simulink model "MPC_sim"  (R2024b)
settings: Solver=FixedStepAuto  StartTime=0.0  StopTime=inf  FixedStep=0.001  RelTol=1e-3  EnableMultiTasking=on
values from neighbouring files (symbols this model uses):
  Ts = 0.01    [MPC.m]    (also in mpc3D.m)
libraries: mpclib x2, px4Sensorslib x2, px4Peripheralslib x1
settings Model: SimulationMode=external  ExtModeTrigDuration=10  Creator=ArriGE66  LastModifiedBy=xippa
settings SolverCC: PositivePriorityOrder=on
settings OptimizationCC: EnhancedBackFolding=on  PassReuseOutputArgsAs=Individual arguments  ZeroExternalMemoryAtStartup=off  ZeroInternalMemoryAtStartup=off  MaxStackSize=64  OptimizeBlockOrder=speed  DifferentSizesBufferReuse=on  OptimizationCustomize=off  EfficientTunableParamExpr=on
settings DebuggingCC: ParameterTunabilityLossMsg=error
settings HardwareCC: ProdBitPerPointer=32  ProdBitPerSizeT=32  ProdBitPerPtrDiffT=32  ProdLargestAtomicInteger=Long  ProdLargestAtomicFloat=Double  ProdWordSize=32  ProdLongLongMode=on  ProdHWDeviceType=ARM Compatible->ARM Cortex
settings SFSimCC: MATLABDynamicMemAlloc=off  SimTargetLang=C++
settings RTWCC: Description=Embedded Coder  SystemTargetFile=ert.tlc  HardwareBoard=PX4 Cube Orange  TemplateMakefile=ert_default_tmf  Toolchain=GNU Tools for PX4 Autopilots  TargetLang=C++  GPUComputeCapability=3.5
settings CodeAppCC: ForceParamTrailComments=on  IgnoreCustomStorageClasses=off  OperatorAnnotations=on  SimulinkDataObjDesc=on  SFDataObjDesc=on  InsertBlockDesc=on
settings ERTTargetCC: SupportVariableSizeSignals=on  ExtMode=on  ExtModeTransport=3  ExtModeStaticAlloc=on  ExtModeStaticAllocSize=1024  ExtModeMexFile=ext_xcp  ExtModeMexArgs=1 COM10 3000000  ExtModeIntrfLevel=Level2 - Open  InlinedParameterPlacement=Hierarchical  DynamicArrayContainerType=coder::array

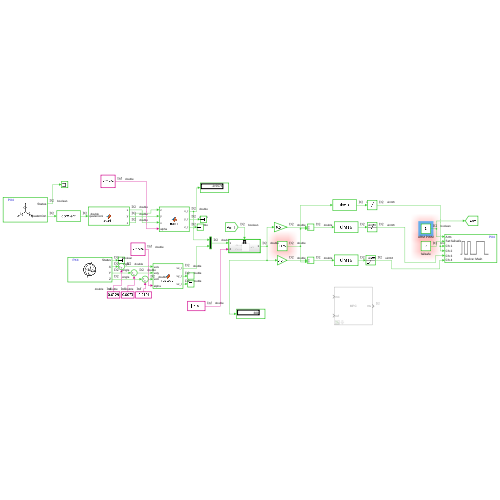
[thumbnail: Simulink's stored preview of the top-level diagram]
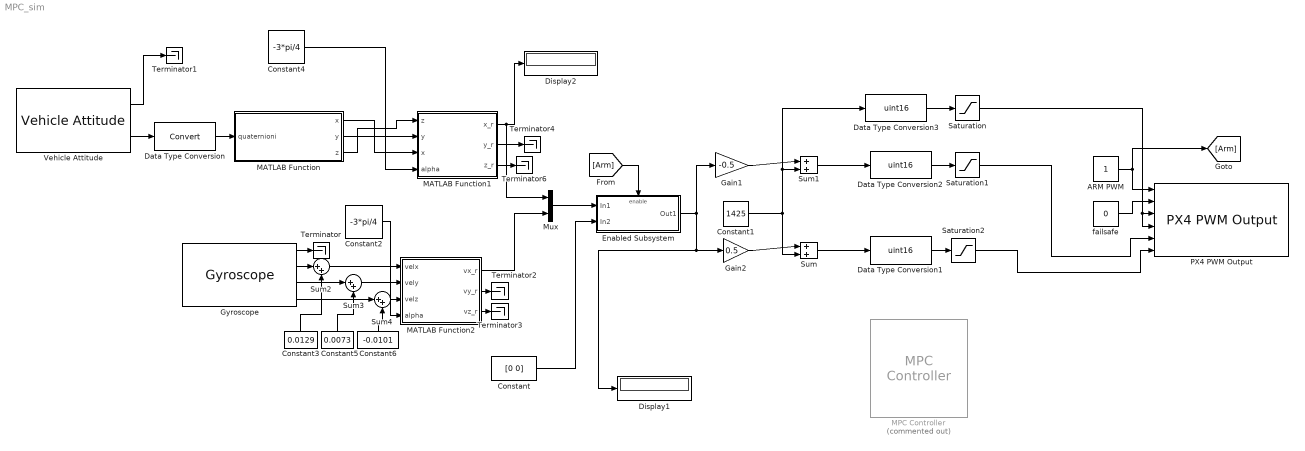
== system MPC_sim ==
  ARM PWM : Constant  OutDataTypeStr=boolean  SampleTime=Ts
  Constant : Constant  Value=[0 0]
  Constant1 : Constant  Value=1425  SampleTime=Ts
  Constant2 : Constant  Value=-3*pi/4
  Constant3 : Constant  Value=0.0129
  Constant4 : Constant  Value=-3*pi/4
  Constant5 : Constant  Value=0.0073
  Constant6 : Constant  Value=-0.0101
  Data Type Conversion : DataTypeConversion  SaturateOnIntegerOverflow=off  RndMeth=Floor
  Data Type Conversion1 : DataTypeConversion  OutDataTypeStr=uint16  SaturateOnIntegerOverflow=off  RndMeth=Floor
  Data Type Conversion2 : DataTypeConversion  OutDataTypeStr=uint16  SaturateOnIntegerOverflow=off  RndMeth=Floor
  Data Type Conversion3 : DataTypeConversion  OutDataTypeStr=uint16  SaturateOnIntegerOverflow=off  RndMeth=Floor
  Display1 : Display
  Display2 : Display
  Enabled Subsystem : Subsystem  TreatAsAtomicUnit=on
  Gain1 : Gain  Gain=-0.5
  Gain2 : Gain  Gain=0.5
  Gyroscope : px4Sensorslib/Gyroscope  uorbTimeStamp=off  BlockingMode=off  BlockTimeout=1e-3  sampleTime=Ts
  MATLAB Function : MATLAB Function  TreatAsAtomicUnit=on
  MATLAB Function1 : MATLAB Function  TreatAsAtomicUnit=on
  MATLAB Function2 : MATLAB Function  TreatAsAtomicUnit=on
  MPC Controller : mpclib/MPC Controller  Commented=on  SCDEnableBlockLinearizationSpecification=on  mpcobj=mpcobj  x0=Init_cond  is_multiple=0  enable_value=0  return_u0=off  updateMPCinCallerWorkspace=on  md_inport=off  mv_inport=off  uref_inport=off  return_cost=off  return_mvseq=off  return_qpstatus=off  return_xseq=off  return_state=off  return_ovseq=off  state_inport=off  umin_inport=off  umax_inport=off  ymin_inport=off  ymax_inport=off  cc_inport=off  ywt_inport=off  uwt_inport=off  duwt_inport=off  rhoeps_inport=off  pm_inport=off  MaximumP=10  HorizonChoice=FixedHorizon  n_ts=0.01  n_p=80  n_mv=1  n_md=0  n_ud=0  n_mo=2  n_uo=0  BlockDataType=double  SampleTimeInherited=off  switch_inport=off
  Mux : Mux  Inputs=2
  PX4 PWM Output : px4Peripheralslib/PX4 PWM Output  pwmDevice=Main  pwmChannel1_=on  pwmChannel2_=on  pwmChannel3_=on  pwmChannel4_=on  pwmChannel5_=off  pwmChannel6_=off  pwmChannel7_=off  pwmChannel8_=off
  Saturation : Saturate  UpperLimit=1800  LowerLimit=1100
  Saturation1 : Saturate  UpperLimit=1800  LowerLimit=1100
  Saturation2 : Saturate  UpperLimit=1800  LowerLimit=1100
  Sum{,1..4} (5 alike) : Sum  Inputs=|++
  Terminator{,1..4,6} (6 alike) : Terminator
  Vehicle Attitude : px4Sensorslib/Vehicle Attitude  rollRate=off  pitchRate=off  yawRate=off  quaternion=on  uorbTimeStamp=off  BlockingMode=off  BlockTimeout=0.001  sampleTime=Ts
  failsafe : Constant  Value=0  OutDataTypeStr=boolean  SampleTime=Ts
  wires:
  Gain1/1 -> Sum1/1
  Gain2/1 -> Sum/1
  Vehicle Attitude/1 -> Terminator1/1
  Vehicle Attitude/2 -> Data Type Conversion/1
  Gyroscope/1 -> Terminator/1
  Gyroscope/3 -> Sum3/1
  Constant2/1 -> MATLAB Function2/4(alpha)
  Gyroscope/2 -> Sum2/1
  Gyroscope/4 -> Sum4/1
  MATLAB Function/1(x) -> MATLAB Function1/3(x)
  MATLAB Function/2(y) -> MATLAB Function1/2(y)
  MATLAB Function/3(z) -> MATLAB Function1/1(z)
  Constant4/1 -> MATLAB Function1/4(alpha)
  Constant1/1 -> Sum1/2, Data Type Conversion3/1, Sum/2
  Sum/1 -> Data Type Conversion1/1
  Sum1/1 -> Data Type Conversion2/1
  Data Type Conversion1/1 -> Saturation2/1
  Data Type Conversion2/1 -> Saturation1/1
  ARM PWM/1 -> PX4 PWM Output/1, [Arm]
  Data Type Conversion3/1 -> Saturation/1
  failsafe/1 -> PX4 PWM Output/2
  MATLAB Function1/1(x_r) -> Display2/1, Mux/1
  MATLAB Function2/1(vx_r) -> Mux/2
  Saturation/1 -> PX4 PWM Output/4, PX4 PWM Output/3
  Saturation2/1 -> PX4 PWM Output/6
  Saturation1/1 -> PX4 PWM Output/5
  Constant5/1 -> Sum3/2
  Constant3/1 -> Sum2/2
  Constant6/1 -> Sum4/2
  Sum2/1 -> MATLAB Function2/1(velx)
  Sum3/1 -> MATLAB Function2/2(vely)
  Sum4/1 -> MATLAB Function2/3(velz)
  MATLAB Function2/2(vy_r) -> Terminator2/1
  MATLAB Function2/3(vz_r) -> Terminator3/1
  MATLAB Function1/2(y_r) -> Terminator4/1
  MATLAB Function1/3(z_r) -> Terminator6/1
  Data Type Conversion/1 -> MATLAB Function/1(quaternioni)
  Mux/1 -> Enabled Subsystem/1(In1)
  Constant/1 -> Enabled Subsystem/2(In2)
  Enabled Subsystem/1(Out1) -> Gain2/1, Display1/1, Gain1/1
  [Arm] -> Enabled Subsystem/Enable

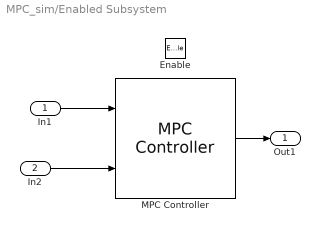
== system MPC_sim/Enabled Subsystem ==
  In1 : Inport
  In2 : Inport  Port=2
  Enable : EnablePort
  MPC Controller : mpclib/MPC Controller  SCDEnableBlockLinearizationSpecification=on  mpcobj=mpcobj  x0=Init_cond  is_multiple=0  enable_value=0  return_u0=off  updateMPCinCallerWorkspace=on  md_inport=off  mv_inport=off  uref_inport=off  return_cost=off  return_mvseq=off  return_qpstatus=off  return_xseq=off  return_state=off  return_ovseq=off  state_inport=off  umin_inport=off  umax_inport=off  ymin_inport=off  ymax_inport=off  cc_inport=off  ywt_inport=off  uwt_inport=off  duwt_inport=off  rhoeps_inport=off  pm_inport=off  MaximumP=10  HorizonChoice=FixedHorizon  n_ts=0.01  n_p=10  n_mv=1  n_md=0  n_ud=0  n_mo=2  n_uo=0  BlockDataType=double  SampleTimeInherited=off  switch_inport=off
  Out1 : Outport
  wires:
  In1/1 -> MPC Controller/1
  In2/1 -> MPC Controller/2
  MPC Controller/1 -> Out1/1

== matlab function MPC_sim/MATLAB Function1 ==
  data: z input; y input; x input; x_r output; alpha input; y_r output; z_r output
function [x_r,y_r,z_r] = ruoto(z,y,x,alpha)
Global_POV = [x y z];
R_z = [cos(alpha), -sin(alpha), 0;
       sin(alpha), cos(alpha), 0;
       0, 0, 1];
LOCALPOV = Global_POV * R_z;
x_r = LOCALPOV(1);
y_r = LOCALPOV(2);
z_r = LOCALPOV(3);
end

== matlab function MPC_sim/MATLAB Function ==
  data: x output; y output; quaternioni input; z output
function [x, y, z] = assetto(quaternioni)
    % Estrazione dei componenti del quaternione
    qw = quaternioni(1);
    qx = quaternioni(2);
    qy = quaternioni(3);
    qz = quaternioni(4);

    % Calcolo degli angoli di Eulero manualmente
    x = atan2(2*(qw*qx + qy*qz), 1 - 2*(qx^2 + qy^2)); % roll
    y = asin(2*(qw*qy - qz*qx));                          % Pitch
    z = atan2(2*(qw*qz + qx*qy), 1 - 2*(qy^2 + qz^2));   % yaw
end

== matlab function MPC_sim/MATLAB Function2 ==
  data: velx input; vely input; velz input; vx_r output; alpha input; vy_r output; vz_r output
function [vx_r, vy_r,vz_r] = ruotovel(velx,vely,velz,alpha)
Global_POV = [velx vely velz];
R_z = [cos(alpha), -sin(alpha), 0;
       sin(alpha), cos(alpha), 0;
       0, 0, 1];
LOCALPOV = Global_POV * R_z;
vx_r = LOCALPOV(1);
vy_r = LOCALPOV(2);
vz_r = LOCALPOV(3);
end
